simulink model "DCMotorSpeedControl"  (R2026b)
settings: Solver=FixedStepDiscrete  StopTime=CL_StopTime  FixedStep=Ts
PreLoadFcn:
  | DCMotorParams;
InitFcn:
  | DCMotorParams;
values from neighbouring files (symbols this model uses):
  PI_Ki = 1/(Plant_K*Spd_Tcl)    (= 0.460405156538)    [DCMotorParams.m]
  PI_Kp = Plant_Tau/(Plant_K*Spd_Tcl)    (= 0.013167587477)    [DCMotorParams.m]
  PI_UMax = 100    [DCMotorParams.m]
  PI_UMin = -100    [DCMotorParams.m]
  Ts = 0.01    [DCMotorParams.m]
libraries: slpidlib x1, simulink x1
settings Model: SILPILModeSetting=veronly  Creator=bence  LastModifiedBy=bence
settings SolverCC: AutoInsertRateTranBlk=on
settings OptimizationCC: DifferentSizesBufferReuse=on  EfficientTunableParamExpr=on  EnhancedBackFolding=on  MaxStackSize=64  OptimizationCustomize=off  OptimizeBlockOrder=speed  PassReuseOutputArgsAs=Individual arguments  RemoveInternalMemoryZeroInit=on  RemoveRootLevelIOMemoryZeroInit=on
settings DebuggingCC: ParameterTunabilityLossMsg=error
settings HardwareCC: ProdHWDeviceType=Atmel->AVR  ProdLargestAtomicFloat=None
settings SFSimCC: MATLABDynamicMemAlloc=off
settings RTWCC: BuildConfiguration=Faster Runs  Description=Embedded Coder  HardwareBoard=Arduino Uno  SystemTargetFile=ert.tlc  TLCOptions=-aInlineSetEventsForThisBaseRateFcn=TLC_FALSE -aSuppressMultiTaskScheduler=TLC_FALSE -aRateBasedStepFcn=1  TemplateMakefile=ert_default_tmf  Toolchain=Arduino AVR
settings CodeAppCC: ForceParamTrailComments=on  IgnoreCustomStorageClasses=off  InsertBlockDesc=on  OperatorAnnotations=on  SFDataObjDesc=on  SimulinkDataObjDesc=on
settings ERTTargetCC: CombineSignalStateStructs=on  ExtMode=on  ExtModeAutomaticAllocSize=off  ExtModeIntrfLevel=Level2 - Open  ExtModeMexFile=ext_xcp  ExtModeStaticAlloc=on  SupportContinuousTime=on  SupportVariableSizeSignals=on

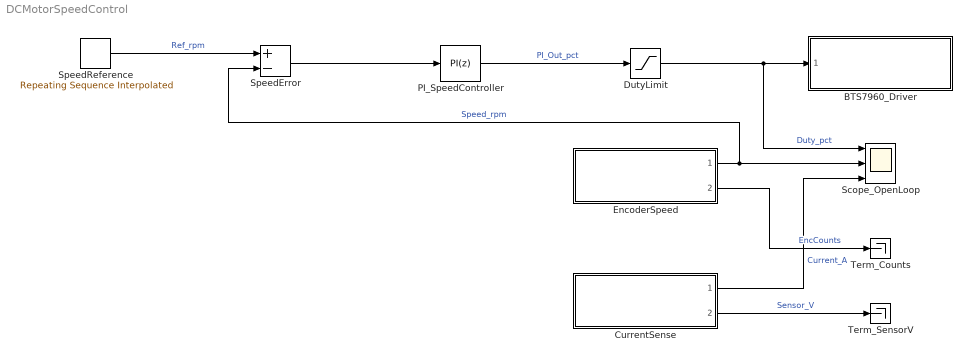
== system DCMotorSpeedControl ==
  BTS7960_Driver : Subsystem  ReferencedSubsystem=DC7960MDriver
  CurrentSense : Subsystem  ReferencedSubsystem=CurrentSense
  DutyLimit : Saturate  UpperLimit=100  LowerLimit=-100
  EncoderSpeed : Subsystem  ReferencedSubsystem=EncoderSpeed
  PI_SpeedController : slpidlib/PID Controller  Controller=PI  Form=Parallel  TimeDomain=Discrete-time  UseExternalTs=off  SampleTime=Ts  IntegratorMethod=Forward Euler  FilterMethod=Forward Euler  ControllerParametersSource=internal  P=PI_Kp  I=PI_Ki  UseKiTs=off  D=0  UseExternalDerivativeSource=off  N=100  UseFilter=on  TunerSelectOption=Transfer Function Based (PID Tuner App)  InitialConditionSource=internal  InitialConditionForIntegrator=0  InitialConditionForFilter=0  DifferentiatorICPrevScaledInput=0  ExternalReset=none  TrackingMode=off  Kt=1  LimitOutput=on  SatLimitsSource=internal  UpperSaturationLimit=PI_UMax  LowerSaturationLimit=PI_UMin  LinearizeAsGain=off  AntiWindupMode=clamping  Kb=1  LimitIntegrator=off  UpperIntegratorSaturationLimit=inf  LowerIntegratorSaturationLimit=-inf  POutMin=[]  POutMax=[]  IOutMin=[]  IOutMax=[]  DOutMin=[]  DOutMax=[]  NOutMin=[]  NOutMax=[]  SumOutMin=[]  SumOutMax=[]  SaturationOutMin=[]  SaturationOutMax=[]  PParamMin=[]  PParamMax=[]  IParamMin=[]  IParamMax=[]  DParamMin=[]  DParamMax=[]  NParamMin=[]  NParamMax=[]  KbParamMin=[]  KbParamMax=[]  KtParamMin=[]  KtParamMax=[]  KbOutMin=[]  KbOutMax=[]  KtOutMin=[]  KtOutMax=[]  IntegratorOutMin=[]  IntegratorOutMax=[]  FilterOutMin=[]  FilterOutMax=[]  SumI1OutMin=[]  SumI1OutMax=[]  SumI2OutMin=[]  SumI2OutMax=[]  SumI3OutMin=[]  SumI3OutMax=[]  SumI4OutMin=[]  SumI4OutMax=[]  SumDOutMin=[]  SumDOutMax=[]  DifferentiatorOutMin=[]  DifferentiatorOutMax=[]  FilterDiffOutCoefMin=[]  FilterDiffOutCoefMax=[]  ReciprocalOutMin=[]  ReciprocalOutMax=[]  SumDenOutMin=[]  SumDenOutMax=[]  SumNumOutMin=[]  SumNumOutMax=[]  DivideOutMin=[]  DivideOutMax=[]  UdiffTsProdOutMin=[]  UdiffTsProdOutMax=[]  NTsProdOutMin=[]  NTsProdOutMax=[]  UintegralTsProdOutMin=[]  UintegralTsProdOutMax=[]  UngainTsProdOutMin=[]  UngainTsProdOutMax=[]  ClampingZeroOutDataTypeStr=Inherit: Inherit via back propagation  ClampingZeroOutMin=[]  ClampingZeroOutMax=[]  FilterDenConstantOutDataTypeStr=Inherit: Inherit via back propagation  FilterDenConstantOutMin=[]  FilterDenConstantOutMax=[]  PCopyOutDataTypeStr=Inherit: Inherit via back propagation  PCopyOutMin=[]  PCopyOutMax=[]  NCopyOutDataTypeStr=Inherit: Inherit via back propagation  NCopyOutMin=[]  NCopyOutMax=[]  IntegratorContinuousStateAttributes=''  IntegratorStateMustResolveToSignalObject=off  IntegratorRTWStateStorageClass=Auto  FilterContinuousStateAttributes=''  FilterStateMustResolveToSignalObject=off  FilterRTWStateStorageClass=Auto  ParallelPVariant=InternalParameters  IdealPVariant=Disabled  IVariant=InternalParameters  DVariant=Disabled  IntegratorVariant=Discrete  SatVariant=Enabled  AWVariant=DiscClampingParallel  PCopyVariant=Disabled  TRVariant=Disabled  FdbkBlocksVariant=Forward  IdealPFdbkVariant=Disabled  SatFdbkVariant=Disabled  DerivativeFilterVariant=Disabled  NVariant=Disabled  NCopyVariant=Disabled_SignalSpec  FilterICVariant=Disabled  IntegratorICVariant=InternalICs  ExternalResetVariant=Disabled  TRSumVariant=Passthrough  SumFdbkVariant=Disabled  SumVariant=Sum_PI  TsampFilterVariant=InternalTs  TsampNgainVariant=Passthrough  TsampIntegralVariant=Disabled_SignalSpec  ExternalSaturationOutDataTypeStr=Inherit: Same as second input  DerivativeSourceVariant=Disabled  PreIntVariant=InternalPreInt
      settings: LibrarySourceBlock=hdlsllib/Discrete/Discrete PID Controller
  Scope_OpenLoop : Scope  NumInputPorts=3
      settings: ActiveDisplayYMinimum=-1863.7162780761719  ActiveDisplayYMaximum=1712.6359558105469
  SpeedError : Sum  Inputs=+-
  SpeedReference : simulink/Sources/Repeating Sequence Interpolated  OutValues=Ref_Values.'  TimeValues=Ref_Time.'  LookUpMeth=Use Input Below  tsamp=Ts  OutMin=[]  OutMax=[]  OutDataTypeStr=double  OutputDataTypeScalingMode=double  OutDataType=fixdt(0,8)  OutScaling=2^-10
  Term_Counts : Terminator
  Term_SensorV : Terminator
  wires:
  CurrentSense/2 -> Term_SensorV/1  "Sensor_V"
  EncoderSpeed/2 -> Term_Counts/1  "EncCounts"
  CurrentSense/1 -> Scope_OpenLoop/3  "Current_A"
  DutyLimit/1 -> BTS7960_Driver/1, Scope_OpenLoop/1  "Duty_pct"
  PI_SpeedController/1 -> DutyLimit/1  "PI_Out_pct"
  SpeedError/1 -> PI_SpeedController/1
  SpeedReference/1 -> SpeedError/1  "Ref_rpm"
  EncoderSpeed/1 -> SpeedError/2, Scope_OpenLoop/2  "Speed_rpm"
